simulink model "test"  (R2022b)
settings: Solver=VariableStepAuto  StartTime=0.0  StopTime=10.0  MaxStep=1e-5  RelTol=1e-3
values from neighbouring files (symbols this model uses):
  Rc = Voc^2 / Poc    (= 5.95521706426)    [Transformer_Performance_Study.m]    (also in data.mat)
  Req = Psc / Isc^2    (= 0.0197785644547)    [Transformer_Performance_Study.m]    (also in data.mat)
  V1 = Voc + 60    (= 221737)    [Transformer_Performance_Study.m]    (also in data.mat)
  Xeq = sqrt(Zeq^2 - Req^2)    [Transformer_Performance_Study.m]    (also in data.mat = 0.0968947815178)
  Xm = Voc / Im    [Transformer_Performance_Study.m]    (also in data.mat = 3.43824617513)
libraries: spsCurrentMeasurementLib x2, spsVoltageMeasurementLib x2, spsACVoltageSourceLib x1, spsGroundLib x1, spsParallelRLCBranchLib x1, spsPowerLib x1, spsSeriesRLCBranchLib x1, spsSeriesRLCLoadLib x1, spsVariableRatioTransformerLib x1, sps_lib x1
settings Model: Creator=moham  LastModifiedBy=moham

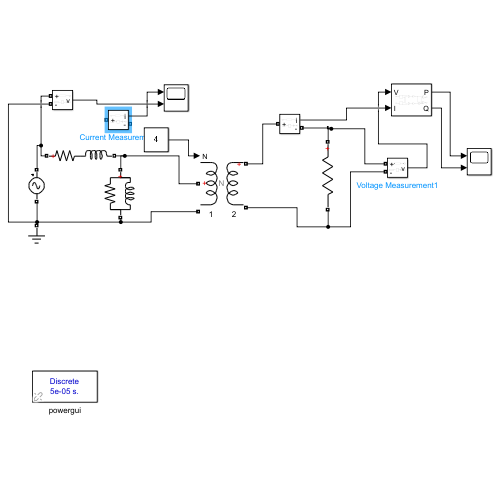
[thumbnail: Simulink's stored preview of the top-level diagram]
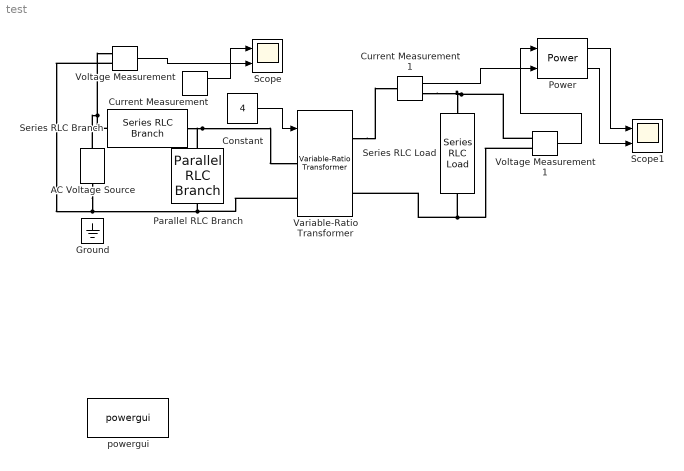
== system test ==
  AC Voltage Source : spsACVoltageSourceLib/AC Voltage Source  Amplitude=(V1)/((2)^(1/2))  Phase=0  Frequency=50  SampleTime=0  Measurements=None  BusType=swing  Pref=10e3  Qref=0  Qmin=-inf  Qmax=+inf
  Constant : Constant  Value=4
  Current Measurement : spsCurrentMeasurementLib/Current Measurement  PhasorSimulation=off  OutputType=Complex  PSBequivalent=0
  Current Measurement1 : spsCurrentMeasurementLib/Current Measurement  PhasorSimulation=off  OutputType=Complex  PSBequivalent=0
  Ground : spsGroundLib/Ground  LConnTagsString=a
  Parallel RLC Branch : spsParallelRLCBranchLib/Parallel RLC Branch  LConnTagsString=a  RConnTagsString=__new0  BranchType=RL  Resistance=Rc  Inductance=Xm/(2*pi*50)  SetiL0=off  InitialCurrent=0  Capacitance=1e-6  Setx0=off  InitialVoltage=0  Measurements=None
  Power : spsPowerLib/Power  Freq=60  Vinit=[1, 0]  Iinit=[1, 0]  Ts=0
  Scope : Scope  NumInputPorts=2
  Scope1 : Scope  NumInputPorts=2
  Series RLC Branch : spsSeriesRLCBranchLib/Series RLC Branch  LConnTagsString=__new0  RConnTagsString=__new0  BranchType=RL  Resistance=Req  Inductance=Xeq/(2*pi*50)  SetiL0=off  InitialCurrent=0  Capacitance=1e-6  Setx0=off  InitialVoltage=0  Measurements=None
  Series RLC Load : spsSeriesRLCLoadLib/Series RLC Load  LConnTagsString=a  RConnTagsString=__new0  NominalVoltage=1000  NominalFrequency=50  ActivePower=2000  InductivePower=0  CapacitivePower=0  Setx0=off  InitialVoltage=0  SetiL0=off  InitialCurrent=0  Measurements=None  LoadType=constant Z
  Variable-Ratio Transformer : spsVariableRatioTransformerLib/Variable-Ratio Transformer
      settings: LibrarySourceBlock=|
      | sps_lib/Passives/Variable-Ratio
      | Transformer
  Voltage Measurement : spsVoltageMeasurementLib/Voltage Measurement  PhasorSimulation=off  OutputType=Complex  PSBequivalent=0
  Voltage Measurement1 : spsVoltageMeasurementLib/Voltage Measurement  PhasorSimulation=off  OutputType=Complex  PSBequivalent=0
  powergui : sps_lib/powergui  Priority=1  SimulationMode=Discrete  SampleTime=50e-6  frequency=60  Iterations=50  frequencyindice=50  Pbase=100e6  ErrMax=1e-4  UnitsV=kV  UnitsW=MW  buscounter=0  FunctionMessages=off  echomessages=off  EnableUseOfTLC=off  CurrentSourceSwitches=off  DisableSnubberDevices=off  DisableRonSwitches=off  DisableVfSwitches=off  DisplayEquations=off  AutomaticDiscreteSolvers=off  SolverType=Tustin/Backward Euler (TBE)  Interpol=off  ExternalGateDelay=off  methode=off  Ts=100  x0status=blocks  SPID=on  SwTol=0  HookPort=off  NonlinearTolerance=1e-4  nMaxIteration=100  ContinueOnMaxIteration=off  RestoreLinks=warning  ResistiveCurrentMeasurement=off  Frange=[0:2:500]  Ylog=off  Xlog=on  ShowGrid=off  save=off  variable=ZData  structure=0  ZoomFFT=off  StartTime=0.0  cycles=1  DisplayStyle=1  fundamental=60  FreqAxis=off  MaxFrequency=1000  frequencyindicesteady=1  RmsSteady=1  display=off
  wires:
  Constant/1 -> Variable-Ratio Transformer/1
  Current Measurement/1 -> Scope/1
  Voltage Measurement/1 -> Scope/2
  Current Measurement1/1 -> Power/2
  Voltage Measurement1/1 -> Power/1
  Power/1 -> Scope1/1
  Power/2 -> Scope1/2
  connections:
  Series RLC Branch/LConn1 -- AC Voltage Source/RConn1 -- Voltage Measurement/LConn1
  AC Voltage Source/LConn1 -- Voltage Measurement/LConn2 -- Variable-Ratio Transformer/LConn2 -- Parallel RLC Branch/RConn1
  Series RLC Branch/RConn1 -- Variable-Ratio Transformer/LConn1 -- Parallel RLC Branch/LConn1
  Voltage Measurement1/LConn1 -- Current Measurement1/RConn1 -- Series RLC Load/LConn1
  Voltage Measurement1/LConn2 -- Variable-Ratio Transformer/RConn2 -- Series RLC Load/RConn1
  Variable-Ratio Transformer/RConn1 -- Current Measurement1/LConn1
